simulink model "AFC_FFNN_trainlm_45_45_45_Nor_July_15"  (R2021a)
settings: Solver=ode15s  StartTime=0.0  StopTime=T  MaxStep=.01  RelTol=1e-3
undefined symbols (not defined in the file): AF_sensor_tol, fault_time, fuel_inj_tol, kappa_tol, MAF_sensor_tol, pump_tol, tau_ww_tol, x_gain, x_offset, y_gain, y_offset
libraries: neural x140
(part 2 of 6)

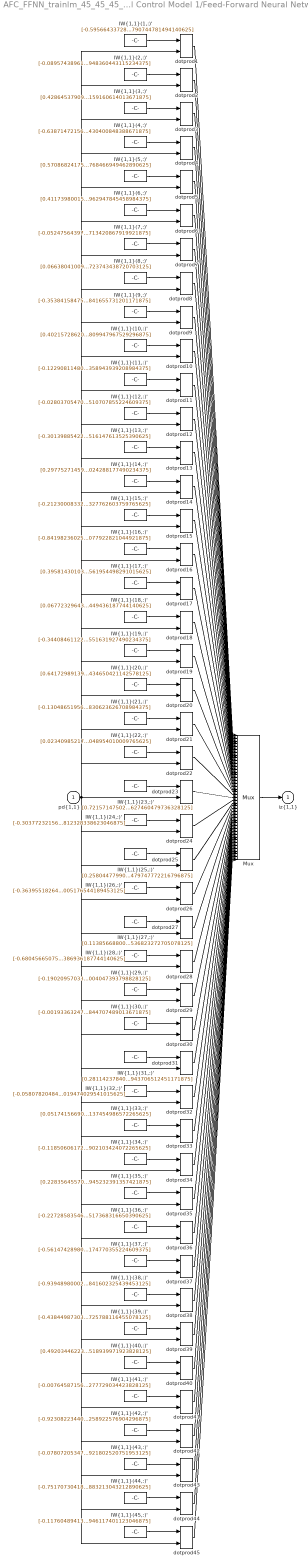
== system AFC_FFNN_trainlm_45_45_45_Nor_July_15/Air Fuel Control Model 1/Feed-Forward Neural Network/Layer 1/IW{1,1} ==
  "pd{1,1}" : Inport  PortDimensions=4
      mask Display: e = 0.06;c1 = [120 230 180]/255;c2 = ([120 230 180]+0)/(256+128);c3 = ([120 230 180]+128)/(256+128);patch([0 1 1 0],[0 0 1 1],c1);patch([0 1 1 1-e 1-e 0+e],[0 0 1 1-e 0+e 0+e],c2);patch([0 0 1 1-e 0+e 0+e],[0 1 1 1-e 1-e 0+e],c3);plot([0 1 1 0 0],[0 0 1 1 0]);
  "IW{1,1}(1,:)'" : Constant  Value=[-0.5956643372825727311692389775998890399932861328125;0.0078851356521167925706095047644339501857757568359375;-0.731583275475554462019545098883099853992462158203125;0.120278687477326062804650064208544790744781494140625]
      mask Display: e = 0.06;c1 = [120 150 230]/255;c2 = ([120 150 230]+0)/383;c3 = ([120 150 230]+128)/383;patch([0 1 1 0],[0 0 1 1],c1);patch([0 1 1 1-e 1-e 0+e],[0 0 1 1-e 0+e 0+e],c2);patch([0 0 1 1-e 0+e 0+e],[0 1 1 1-e 1-e 0+e],c3);plot([0 1 1 0 0],[0 0 1 1 0]);disp('Weights');
  "IW{1,1}(10,:)'" : Constant  Value=[0.40215728620280477567661137072718702256679534912109375;0.215024407178198206924690794039634056389331817626953125;0.2250727041009067119770037379566929303109645843505859375;0.435264136292866143929103373011457733809947967529296875]
      mask Display: e = 0.06;c1 = [120 150 230]/255;c2 = ([120 150 230]+0)/383;c3 = ([120 150 230]+128)/383;patch([0 1 1 0],[0 0 1 1],c1);patch([0 1 1 1-e 1-e 0+e],[0 0 1 1-e 0+e 0+e],c2);patch([0 0 1 1-e 0+e 0+e],[0 1 1 1-e 1-e 0+e],c3);plot([0 1 1 0 0],[0 0 1 1 0]);disp('Weights');
  "IW{1,1}(11,:)'" : Constant  Value=[-0.1229081148035984227817607461474835872650146484375;-0.69490483860332563637030034442432224750518798828125;-0.453944678170142612572135476511903107166290283203125;0.0741787341554722701175705878995358943939208984375]
      mask Display: e = 0.06;c1 = [120 150 230]/255;c2 = ([120 150 230]+0)/383;c3 = ([120 150 230]+128)/383;patch([0 1 1 0],[0 0 1 1],c1);patch([0 1 1 1-e 1-e 0+e],[0 0 1 1-e 0+e 0+e],c2);patch([0 0 1 1-e 0+e 0+e],[0 1 1 1-e 1-e 0+e],c3);plot([0 1 1 0 0],[0 0 1 1 0]);disp('Weights');
  "IW{1,1}(12,:)'" : Constant  Value=[-0.0280370547053085221456125708527906681410968303680419921875;0.0235006232351334908015072500120368204079568386077880859375;-0.99679528598227229441164354284410364925861358642578125;-0.139054055078011662427428518640226684510707855224609375]
      mask Display: e = 0.06;c1 = [120 150 230]/255;c2 = ([120 150 230]+0)/383;c3 = ([120 150 230]+128)/383;patch([0 1 1 0],[0 0 1 1],c1);patch([0 1 1 1-e 1-e 0+e],[0 0 1 1-e 0+e 0+e],c2);patch([0 0 1 1-e 0+e 0+e],[0 1 1 1-e 1-e 0+e],c3);plot([0 1 1 0 0],[0 0 1 1 0]);disp('Weights');
  "IW{1,1}(13,:)'" : Constant  Value=[-0.301398854224746604035800601195660419762134552001953125;0.283042849370989169077716951505863107740879058837890625;0.052267715740464924800701140839009894989430904388427734375;-0.1897669659253120588715546546154655516147613525390625]
      mask Display: e = 0.06;c1 = [120 150 230]/255;c2 = ([120 150 230]+0)/383;c3 = ([120 150 230]+128)/383;patch([0 1 1 0],[0 0 1 1],c1);patch([0 1 1 1-e 1-e 0+e],[0 0 1 1-e 0+e 0+e],c2);patch([0 0 1 1-e 0+e 0+e],[0 1 1 1-e 1-e 0+e],c3);plot([0 1 1 0 0],[0 0 1 1 0]);disp('Weights');
  "IW{1,1}(14,:)'" : Constant  Value=[0.2977527145915799255959655056358315050601959228515625;0.389318770656627621828960172933875583112239837646484375;0.293057371345684547492282945313490927219390869140625;0.2813997438522173322184016797109507024288177490234375]
      mask Display: e = 0.06;c1 = [120 150 230]/255;c2 = ([120 150 230]+0)/383;c3 = ([120 150 230]+128)/383;patch([0 1 1 0],[0 0 1 1],c1);patch([0 1 1 1-e 1-e 0+e],[0 0 1 1-e 0+e 0+e],c2);patch([0 0 1 1-e 0+e 0+e],[0 1 1 1-e 1-e 0+e],c3);plot([0 1 1 0 0],[0 0 1 1 0]);disp('Weights');
  "IW{1,1}(15,:)'" : Constant  Value=[-0.21230008332540395432630475625046528875827789306640625;0.68052922423117545580595333376550115644931793212890625;1.129196089459527652110182316391728818416595458984375;0.38175478396998008268070634585455991327762603759765625]
      mask Display: e = 0.06;c1 = [120 150 230]/255;c2 = ([120 150 230]+0)/383;c3 = ([120 150 230]+128)/383;patch([0 1 1 0],[0 0 1 1],c1);patch([0 1 1 1-e 1-e 0+e],[0 0 1 1-e 0+e 0+e],c2);patch([0 0 1 1-e 0+e 0+e],[0 1 1 1-e 1-e 0+e],c3);plot([0 1 1 0 0],[0 0 1 1 0]);disp('Weights');
  "IW{1,1}(16,:)'" : Constant  Value=[-0.8419823602587410693587344212573952972888946533203125;-0.683631419962078101804081597947515547275543212890625;0.136479567974448823264310703962109982967376708984375;0.424886858909423903440938374842517077922821044921875]
      mask Display: e = 0.06;c1 = [120 150 230]/255;c2 = ([120 150 230]+0)/383;c3 = ([120 150 230]+128)/383;patch([0 1 1 0],[0 0 1 1],c1);patch([0 1 1 1-e 1-e 0+e],[0 0 1 1-e 0+e 0+e],c2);patch([0 0 1 1-e 0+e 0+e],[0 1 1 1-e 1-e 0+e],c3);plot([0 1 1 0 0],[0 0 1 1 0]);disp('Weights');
  "IW{1,1}(17,:)'" : Constant  Value=[0.39581430103202530634831646239035762846469879150390625;0.04913474719346826169452668864323641173541545867919921875;-0.37189361256331088245730143171385861933231353759765625;0.0937071221445386071113858861281187273561954498291015625]
      mask Display: e = 0.06;c1 = [120 150 230]/255;c2 = ([120 150 230]+0)/383;c3 = ([120 150 230]+128)/383;patch([0 1 1 0],[0 0 1 1],c1);patch([0 1 1 1-e 1-e 0+e],[0 0 1 1-e 0+e 0+e],c2);patch([0 0 1 1-e 0+e 0+e],[0 1 1 1-e 1-e 0+e],c3);plot([0 1 1 0 0],[0 0 1 1 0]);disp('Weights');
  "IW{1,1}(18,:)'" : Constant  Value=[0.067723296434411162092459335326566360890865325927734375;0.0782261872747194442201390529589843936264514923095703125;-0.7782064126921157676264328983961604535579681396484375;0.66151523134186407393286799560883082449436187744140625]
      mask Display: e = 0.06;c1 = [120 150 230]/255;c2 = ([120 150 230]+0)/383;c3 = ([120 150 230]+128)/383;patch([0 1 1 0],[0 0 1 1],c1);patch([0 1 1 1-e 1-e 0+e],[0 0 1 1-e 0+e 0+e],c2);patch([0 0 1 1-e 0+e 0+e],[0 1 1 1-e 1-e 0+e],c3);plot([0 1 1 0 0],[0 0 1 1 0]);disp('Weights');
  "IW{1,1}(19,:)'" : Constant  Value=[-0.34408461122719469216235665953718125820159912109375;-0.727276266717437724906858420581556856632232666015625;-0.3469464521698870651533752607065252959728240966796875;-0.8895237546480083690170204135938547551631927490234375]
      mask Display: e = 0.06;c1 = [120 150 230]/255;c2 = ([120 150 230]+0)/383;c3 = ([120 150 230]+128)/383;patch([0 1 1 0],[0 0 1 1],c1);patch([0 1 1 1-e 1-e 0+e],[0 0 1 1-e 0+e 0+e],c2);patch([0 0 1 1-e 0+e 0+e],[0 1 1 1-e 1-e 0+e],c3);plot([0 1 1 0 0],[0 0 1 1 0]);disp('Weights');
  "IW{1,1}(2,:)'" : Constant  Value=[-0.0895743896153724517006367022986523807048797607421875;-0.4974994059611235197593259727000258862972259521484375;-0.556921490563318410949023018474690616130828857421875;-0.1468395671085696019275701473816297948360443115234375]
      mask Display: e = 0.06;c1 = [120 150 230]/255;c2 = ([120 150 230]+0)/383;c3 = ([120 150 230]+128)/383;patch([0 1 1 0],[0 0 1 1],c1);patch([0 1 1 1-e 1-e 0+e],[0 0 1 1-e 0+e 0+e],c2);patch([0 0 1 1-e 0+e 0+e],[0 1 1 1-e 1-e 0+e],c3);plot([0 1 1 0 0],[0 0 1 1 0]);disp('Weights');
  "IW{1,1}(20,:)'" : Constant  Value=[0.64172989139603620056817590011633001267910003662109375;0.241314326391462496967932338520768098533153533935546875;-0.5964552046849258548633088139467872679233551025390625;0.155516258518920758024961514820461161434650421142578125]
      mask Display: e = 0.06;c1 = [120 150 230]/255;c2 = ([120 150 230]+0)/383;c3 = ([120 150 230]+128)/383;patch([0 1 1 0],[0 0 1 1],c1);patch([0 1 1 1-e 1-e 0+e],[0 0 1 1-e 0+e 0+e],c2);patch([0 0 1 1-e 0+e 0+e],[0 1 1 1-e 1-e 0+e],c3);plot([0 1 1 0 0],[0 0 1 1 0]);disp('Weights');
  "IW{1,1}(21,:)'" : Constant  Value=[-0.130486519560841729425959556465386413037776947021484375;0.23962567672372758753596144742914475500583648681640625;1.2471840349032419226205092854797840118408203125;-0.217739378918231751836032117353170178830623626708984375]
      mask Display: e = 0.06;c1 = [120 150 230]/255;c2 = ([120 150 230]+0)/383;c3 = ([120 150 230]+128)/383;patch([0 1 1 0],[0 0 1 1],c1);patch([0 1 1 1-e 1-e 0+e],[0 0 1 1-e 0+e 0+e],c2);patch([0 0 1 1-e 0+e 0+e],[0 1 1 1-e 1-e 0+e],c3);plot([0 1 1 0 0],[0 0 1 1 0]);disp('Weights');
  "IW{1,1}(22,:)'" : Constant  Value=[0.0234098521776516139969448460078638163395226001739501953125;0.01181668668611625915010332477095289505086839199066162109375;0.2319172972597932369520634665605030022561550140380859375;0.053573417723569195791899488767739967443048954010009765625]
      mask Display: e = 0.06;c1 = [120 150 230]/255;c2 = ([120 150 230]+0)/383;c3 = ([120 150 230]+128)/383;patch([0 1 1 0],[0 0 1 1],c1);patch([0 1 1 1-e 1-e 0+e],[0 0 1 1-e 0+e 0+e],c2);patch([0 0 1 1-e 0+e 0+e],[0 1 1 1-e 1-e 0+e],c3);plot([0 1 1 0 0],[0 0 1 1 0]);disp('Weights');
  "IW{1,1}(23,:)'" : Constant  Value=[0.7215714750234367702574900249601341784000396728515625;-0.16108688740140753026253150892443954944610595703125;-0.2450954091114052602051742724142968654632568359375;-0.8883730723524536632140780056943185627460479736328125]
      mask Display: e = 0.06;c1 = [120 150 230]/255;c2 = ([120 150 230]+0)/383;c3 = ([120 150 230]+128)/383;patch([0 1 1 0],[0 0 1 1],c1);patch([0 1 1 1-e 1-e 0+e],[0 0 1 1-e 0+e 0+e],c2);patch([0 0 1 1-e 0+e 0+e],[0 1 1 1-e 1-e 0+e],c3);plot([0 1 1 0 0],[0 0 1 1 0]);disp('Weights');
  "IW{1,1}(24,:)'" : Constant  Value=[-0.303772321561371960729758257002686150372028350830078125;-0.13663066884064811734589284242247231304645538330078125;0.28666251978549073253788037618505768477916717529296875;0.0872318977607193513090777514662477187812328338623046875]
      mask Display: e = 0.06;c1 = [120 150 230]/255;c2 = ([120 150 230]+0)/383;c3 = ([120 150 230]+128)/383;patch([0 1 1 0],[0 0 1 1],c1);patch([0 1 1 1-e 1-e 0+e],[0 0 1 1-e 0+e 0+e],c2);patch([0 0 1 1-e 0+e 0+e],[0 1 1 1-e 1-e 0+e],c3);plot([0 1 1 0 0],[0 0 1 1 0]);disp('Weights');
  "IW{1,1}(25,:)'" : Constant  Value=[0.25804477990530061415341833708225749433040618896484375;-0.1588247856223685416932056568839470855891704559326171875;-0.9527621246937447718750036074197851121425628662109375;0.342543129651466660146041931511717848479747772216796875]
      mask Display: e = 0.06;c1 = [120 150 230]/255;c2 = ([120 150 230]+0)/383;c3 = ([120 150 230]+128)/383;patch([0 1 1 0],[0 0 1 1],c1);patch([0 1 1 1-e 1-e 0+e],[0 0 1 1-e 0+e 0+e],c2);patch([0 0 1 1-e 0+e 0+e],[0 1 1 1-e 1-e 0+e],c3);plot([0 1 1 0 0],[0 0 1 1 0]);disp('Weights');
  "IW{1,1}(26,:)'" : Constant  Value=[-0.3639551826419198388151698964065872132778167724609375;-0.954934179958911055763337571988813579082489013671875;0.9311051108874803805548481250298209488391876220703125;-0.2415869542128252778212527118739672005176544189453125]
      mask Display: e = 0.06;c1 = [120 150 230]/255;c2 = ([120 150 230]+0)/383;c3 = ([120 150 230]+128)/383;patch([0 1 1 0],[0 0 1 1],c1);patch([0 1 1 1-e 1-e 0+e],[0 0 1 1-e 0+e 0+e],c2);patch([0 0 1 1-e 0+e 0+e],[0 1 1 1-e 1-e 0+e],c3);plot([0 1 1 0 0],[0 0 1 1 0]);disp('Weights');
  "IW{1,1}(27,:)'" : Constant  Value=[0.113856688004887851572988211046322248876094818115234375;0.156682594473692093917094325661309994757175445556640625;0.404541877953054129779530967425671406090259552001953125;0.3243492455387972928093631708179600536823272705078125]
      mask Display: e = 0.06;c1 = [120 150 230]/255;c2 = ([120 150 230]+0)/383;c3 = ([120 150 230]+128)/383;patch([0 1 1 0],[0 0 1 1],c1);patch([0 1 1 1-e 1-e 0+e],[0 0 1 1-e 0+e 0+e],c2);patch([0 0 1 1-e 0+e 0+e],[0 1 1 1-e 1-e 0+e],c3);plot([0 1 1 0 0],[0 0 1 1 0]);disp('Weights');
  "IW{1,1}(28,:)'" : Constant  Value=[-0.6804566507554359322540449284133501350879669189453125;-0.9876086455192980562145521616912446916103363037109375;-0.4386537506745231684845975905773229897022247314453125;-0.5337541635500218095700120102264918386936187744140625]
      mask Display: e = 0.06;c1 = [120 150 230]/255;c2 = ([120 150 230]+0)/383;c3 = ([120 150 230]+128)/383;patch([0 1 1 0],[0 0 1 1],c1);patch([0 1 1 1-e 1-e 0+e],[0 0 1 1-e 0+e 0+e],c2);patch([0 0 1 1-e 0+e 0+e],[0 1 1 1-e 1-e 0+e],c3);plot([0 1 1 0 0],[0 0 1 1 0]);disp('Weights');
  "IW{1,1}(29,:)'" : Constant  Value=[-0.19020957033060648111444379537715576589107513427734375;0.0103510998057852292297820184785450692288577556610107421875;2.514854966736393304671537407557480037212371826171875;0.16321702287675876608119551747222431004047393798828125]
      mask Display: e = 0.06;c1 = [120 150 230]/255;c2 = ([120 150 230]+0)/383;c3 = ([120 150 230]+128)/383;patch([0 1 1 0],[0 0 1 1],c1);patch([0 1 1 1-e 1-e 0+e],[0 0 1 1-e 0+e 0+e],c2);patch([0 0 1 1-e 0+e 0+e],[0 1 1 1-e 1-e 0+e],c3);plot([0 1 1 0 0],[0 0 1 1 0]);disp('Weights');
  "IW{1,1}(3,:)'" : Constant  Value=[0.4286453790909512395757019476150162518024444580078125;0.33552739865496128413013821045751683413982391357421875;-0.2115595154244242770413819698660518042743206024169921875;-0.55043277454292194317275743742357008159160614013671875]
      mask Display: e = 0.06;c1 = [120 150 230]/255;c2 = ([120 150 230]+0)/383;c3 = ([120 150 230]+128)/383;patch([0 1 1 0],[0 0 1 1],c1);patch([0 1 1 1-e 1-e 0+e],[0 0 1 1-e 0+e 0+e],c2);patch([0 0 1 1-e 0+e 0+e],[0 1 1 1-e 1-e 0+e],c3);plot([0 1 1 0 0],[0 0 1 1 0]);disp('Weights');
  "IW{1,1}(30,:)'" : Constant  Value=[-0.00193363247180133868141638231463730335235595703125;0.1267069804364975293964334923657588660717010498046875;0.1556430626833267272246530410484410822391510009765625;-0.548593431939991216239604909787885844707489013671875]
      mask Display: e = 0.06;c1 = [120 150 230]/255;c2 = ([120 150 230]+0)/383;c3 = ([120 150 230]+128)/383;patch([0 1 1 0],[0 0 1 1],c1);patch([0 1 1 1-e 1-e 0+e],[0 0 1 1-e 0+e 0+e],c2);patch([0 0 1 1-e 0+e 0+e],[0 1 1 1-e 1-e 0+e],c3);plot([0 1 1 0 0],[0 0 1 1 0]);disp('Weights');
  "IW{1,1}(31,:)'" : Constant  Value=[0.2811423784052606844596766677568666636943817138671875;0.57790938879531894567520566852181218564510345458984375;-0.9063653540192044832934925580048002302646636962890625;0.5131888068818895032308091685990802943706512451171875]
      mask Display: e = 0.06;c1 = [120 150 230]/255;c2 = ([120 150 230]+0)/383;c3 = ([120 150 230]+128)/383;patch([0 1 1 0],[0 0 1 1],c1);patch([0 1 1 1-e 1-e 0+e],[0 0 1 1-e 0+e 0+e],c2);patch([0 0 1 1-e 0+e 0+e],[0 1 1 1-e 1-e 0+e],c3);plot([0 1 1 0 0],[0 0 1 1 0]);disp('Weights');
  "IW{1,1}(32,:)'" : Constant  Value=[-0.058078204842097129467770599831055733375251293182373046875;-0.001563164818252172315327097606996176182292401790618896484375;0.82613033699437432577639128794544376432895660400390625;0.1453053847708275780892250850229174830019474029541015625]
      mask Display: e = 0.06;c1 = [120 150 230]/255;c2 = ([120 150 230]+0)/383;c3 = ([120 150 230]+128)/383;patch([0 1 1 0],[0 0 1 1],c1);patch([0 1 1 1-e 1-e 0+e],[0 0 1 1-e 0+e 0+e],c2);patch([0 0 1 1-e 0+e 0+e],[0 1 1 1-e 1-e 0+e],c3);plot([0 1 1 0 0],[0 0 1 1 0]);disp('Weights');
  "IW{1,1}(33,:)'" : Constant  Value=[0.05174156690815133463612340847248560748994350433349609375;0.417236200443662996750759930364438332617282867431640625;0.28576353561735334807281105895526707172393798828125;-0.2301783314639698208026175052509643137454986572265625]
      mask Display: e = 0.06;c1 = [120 150 230]/255;c2 = ([120 150 230]+0)/383;c3 = ([120 150 230]+128)/383;patch([0 1 1 0],[0 0 1 1],c1);patch([0 1 1 1-e 1-e 0+e],[0 0 1 1-e 0+e 0+e],c2);patch([0 0 1 1-e 0+e 0+e],[0 1 1 1-e 1-e 0+e],c3);plot([0 1 1 0 0],[0 0 1 1 0]);disp('Weights');
  "IW{1,1}(34,:)'" : Constant  Value=[-0.11850606172833634543994918431053520180284976959228515625;0.64849251750362368884594843621016480028629302978515625;-0.66071595290289197865973847001441754400730133056640625;-0.08370208249480794171493158728480921126902103424072265625]
      mask Display: e = 0.06;c1 = [120 150 230]/255;c2 = ([120 150 230]+0)/383;c3 = ([120 150 230]+128)/383;patch([0 1 1 0],[0 0 1 1],c1);patch([0 1 1 1-e 1-e 0+e],[0 0 1 1-e 0+e 0+e],c2);patch([0 0 1 1-e 0+e 0+e],[0 1 1 1-e 1-e 0+e],c3);plot([0 1 1 0 0],[0 0 1 1 0]);disp('Weights');
  "IW{1,1}(35,:)'" : Constant  Value=[0.22835645570773610568693356981384567916393280029296875;-0.54905905338665250692287145284353755414485931396484375;-0.89228427011588318240598027841770090162754058837890625;0.1158953695663818006522660652990452945232391357421875]
      mask Display: e = 0.06;c1 = [120 150 230]/255;c2 = ([120 150 230]+0)/383;c3 = ([120 150 230]+128)/383;patch([0 1 1 0],[0 0 1 1],c1);patch([0 1 1 1-e 1-e 0+e],[0 0 1 1-e 0+e 0+e],c2);patch([0 0 1 1-e 0+e 0+e],[0 1 1 1-e 1-e 0+e],c3);plot([0 1 1 0 0],[0 0 1 1 0]);disp('Weights');
  "IW{1,1}(36,:)'" : Constant  Value=[-0.2272858354609279540881061620893888175487518310546875;-0.4763666279626981303607635709340684115886688232421875;0.51951620528753483796435830299742519855499267578125;-0.564515386968702959080701475613750517368316650390625]
      mask Display: e = 0.06;c1 = [120 150 230]/255;c2 = ([120 150 230]+0)/383;c3 = ([120 150 230]+128)/383;patch([0 1 1 0],[0 0 1 1],c1);patch([0 1 1 1-e 1-e 0+e],[0 0 1 1-e 0+e 0+e],c2);patch([0 0 1 1-e 0+e 0+e],[0 1 1 1-e 1-e 0+e],c3);plot([0 1 1 0 0],[0 0 1 1 0]);disp('Weights');
  "IW{1,1}(37,:)'" : Constant  Value=[-0.5614742898029103645995974147808738052845001220703125;-0.29126643634214133271598257124423980712890625;0.152044548675759561007225784123875200748443603515625;-0.59448016906409151260959333740174770355224609375]
      mask Display: e = 0.06;c1 = [120 150 230]/255;c2 = ([120 150 230]+0)/383;c3 = ([120 150 230]+128)/383;patch([0 1 1 0],[0 0 1 1],c1);patch([0 1 1 1-e 1-e 0+e],[0 0 1 1-e 0+e 0+e],c2);patch([0 0 1 1-e 0+e 0+e],[0 1 1 1-e 1-e 0+e],c3);plot([0 1 1 0 0],[0 0 1 1 0]);disp('Weights');
  "IW{1,1}(38,:)'" : Constant  Value=[-0.939489800028924459951440439908765256404876708984375;0.4051451785018820306305542544578202068805694580078125;-0.861338665941364656220002871123142540454864501953125;-0.52987044420598294891533441841602325439453125]
      mask Display: e = 0.06;c1 = [120 150 230]/255;c2 = ([120 150 230]+0)/383;c3 = ([120 150 230]+128)/383;patch([0 1 1 0],[0 0 1 1],c1);patch([0 1 1 1-e 1-e 0+e],[0 0 1 1-e 0+e 0+e],c2);patch([0 0 1 1-e 0+e 0+e],[0 1 1 1-e 1-e 0+e],c3);plot([0 1 1 0 0],[0 0 1 1 0]);disp('Weights');
  "IW{1,1}(39,:)'" : Constant  Value=[-0.438449873032815184981103584505035541951656341552734375;0.82358882068447314406256509755621664226055145263671875;-0.054224785744120963804082435899545089341700077056884765625;0.52110169311764586996815751263056881725788116455078125]
      mask Display: e = 0.06;c1 = [120 150 230]/255;c2 = ([120 150 230]+0)/383;c3 = ([120 150 230]+128)/383;patch([0 1 1 0],[0 0 1 1],c1);patch([0 1 1 1-e 1-e 0+e],[0 0 1 1-e 0+e 0+e],c2);patch([0 0 1 1-e 0+e 0+e],[0 1 1 1-e 1-e 0+e],c3);plot([0 1 1 0 0],[0 0 1 1 0]);disp('Weights');
  "IW{1,1}(4,:)'" : Constant  Value=[-0.6387147215604758176965560778626240789890289306640625;-0.1557107718810311070001262123696506023406982421875;-0.64377405270552490179625237942673265933990478515625;-0.8954322416204518741977835816214792430400848388671875]
      mask Display: e = 0.06;c1 = [120 150 230]/255;c2 = ([120 150 230]+0)/383;c3 = ([120 150 230]+128)/383;patch([0 1 1 0],[0 0 1 1],c1);patch([0 1 1 1-e 1-e 0+e],[0 0 1 1-e 0+e 0+e],c2);patch([0 0 1 1-e 0+e 0+e],[0 1 1 1-e 1-e 0+e],c3);plot([0 1 1 0 0],[0 0 1 1 0]);disp('Weights');
  "IW{1,1}(40,:)'" : Constant  Value=[0.492034462236722702765945314240525476634502410888671875;-0.1777275222817087663162993749210727401077747344970703125;0.0099231706383438623986226190254456014372408390045166015625;-0.5146204597120729307135889030178077518939971923828125]
      mask Display: e = 0.06;c1 = [120 150 230]/255;c2 = ([120 150 230]+0)/383;c3 = ([120 150 230]+128)/383;patch([0 1 1 0],[0 0 1 1],c1);patch([0 1 1 1-e 1-e 0+e],[0 0 1 1-e 0+e 0+e],c2);patch([0 0 1 1-e 0+e 0+e],[0 1 1 1-e 1-e 0+e],c3);plot([0 1 1 0 0],[0 0 1 1 0]);disp('Weights');
  "IW{1,1}(41,:)'" : Constant  Value=[-0.007645871561652416679988331082995500764809548854827880859375;0.035310008323311013744838504635481513105332851409912109375;0.669218883200376257747166164335794746875762939453125;-0.29644770762242089734428418523748405277729034423828125]
      mask Display: e = 0.06;c1 = [120 150 230]/255;c2 = ([120 150 230]+0)/383;c3 = ([120 150 230]+128)/383;patch([0 1 1 0],[0 0 1 1],c1);patch([0 1 1 1-e 1-e 0+e],[0 0 1 1-e 0+e 0+e],c2);patch([0 0 1 1-e 0+e 0+e],[0 1 1 1-e 1-e 0+e],c3);plot([0 1 1 0 0],[0 0 1 1 0]);disp('Weights');
  "IW{1,1}(42,:)'" : Constant  Value=[-0.9230822344099307574794011088670231401920318603515625;0.0345640338353359055645341868512332439422607421875;-0.8821807032780721868903128779493272304534912109375;-0.016831332291136202883308214950375258922576904296875]
      mask Display: e = 0.06;c1 = [120 150 230]/255;c2 = ([120 150 230]+0)/383;c3 = ([120 150 230]+128)/383;patch([0 1 1 0],[0 0 1 1],c1);patch([0 1 1 1-e 1-e 0+e],[0 0 1 1-e 0+e 0+e],c2);patch([0 0 1 1-e 0+e 0+e],[0 1 1 1-e 1-e 0+e],c3);plot([0 1 1 0 0],[0 0 1 1 0]);disp('Weights');
  "IW{1,1}(43,:)'" : Constant  Value=[-0.0780720534746517369484308801474981009960174560546875;-0.76974465630501498480953159742057323455810546875;0.1214981365683154290735501490416936576366424560546875;-0.54355568559331590705596681800670921802520751953125]
      mask Display: e = 0.06;c1 = [120 150 230]/255;c2 = ([120 150 230]+0)/383;c3 = ([120 150 230]+128)/383;patch([0 1 1 0],[0 0 1 1],c1);patch([0 1 1 1-e 1-e 0+e],[0 0 1 1-e 0+e 0+e],c2);patch([0 0 1 1-e 0+e 0+e],[0 1 1 1-e 1-e 0+e],c3);plot([0 1 1 0 0],[0 0 1 1 0]);disp('Weights');
  "IW{1,1}(44,:)'" : Constant  Value=[-0.751707304187491320845992959220893681049346923828125;0.198396436014707688855196465738117694854736328125;0.7254043262583362849937884675455279648303985595703125;-0.918083848242825073526773849152959883213043212890625]
      mask Display: e = 0.06;c1 = [120 150 230]/255;c2 = ([120 150 230]+0)/383;c3 = ([120 150 230]+128)/383;patch([0 1 1 0],[0 0 1 1],c1);patch([0 1 1 1-e 1-e 0+e],[0 0 1 1-e 0+e 0+e],c2);patch([0 0 1 1-e 0+e 0+e],[0 1 1 1-e 1-e 0+e],c3);plot([0 1 1 0 0],[0 0 1 1 0]);disp('Weights');
  "IW{1,1}(45,:)'" : Constant  Value=[-0.11760489413344958620211144761924515478312969207763671875;-0.06724246508251256748689428377474541775882244110107421875;1.716790267288401228285010802210308611392974853515625;0.138135284928623203182240786190959624946117401123046875]
      mask Display: e = 0.06;c1 = [120 150 230]/255;c2 = ([120 150 230]+0)/383;c3 = ([120 150 230]+128)/383;patch([0 1 1 0],[0 0 1 1],c1);patch([0 1 1 1-e 1-e 0+e],[0 0 1 1-e 0+e 0+e],c2);patch([0 0 1 1-e 0+e 0+e],[0 1 1 1-e 1-e 0+e],c3);plot([0 1 1 0 0],[0 0 1 1 0]);disp('Weights');
  "IW{1,1}(5,:)'" : Constant  Value=[0.57086824175524986113572367685264907777309417724609375;0.42698472150594624086039630128652788698673248291015625;-0.911692582119400629636629673768766224384307861328125;0.343660323975889137049222199493669904768466949462890625]
      mask Display: e = 0.06;c1 = [120 150 230]/255;c2 = ([120 150 230]+0)/383;c3 = ([120 150 230]+128)/383;patch([0 1 1 0],[0 0 1 1],c1);patch([0 1 1 1-e 1-e 0+e],[0 0 1 1-e 0+e 0+e],c2);patch([0 0 1 1-e 0+e 0+e],[0 1 1 1-e 1-e 0+e],c3);plot([0 1 1 0 0],[0 0 1 1 0]);disp('Weights');
  "IW{1,1}(6,:)'" : Constant  Value=[0.411739800154247548302777204298763535916805267333984375;0.422359992132983197432594124620663933455944061279296875;0.87224581114104549062204796427977271378040313720703125;0.509079625495759469089307458489201962947845458984375]
      mask Display: e = 0.06;c1 = [120 150 230]/255;c2 = ([120 150 230]+0)/383;c3 = ([120 150 230]+128)/383;patch([0 1 1 0],[0 0 1 1],c1);patch([0 1 1 1-e 1-e 0+e],[0 0 1 1-e 0+e 0+e],c2);patch([0 0 1 1-e 0+e 0+e],[0 1 1 1-e 1-e 0+e],c3);plot([0 1 1 0 0],[0 0 1 1 0]);disp('Weights');
  "IW{1,1}(7,:)'" : Constant  Value=[-0.052475643970241188374092899948664125986397266387939453125;-0.00307760460118986813038421956889578723348677158355712890625;0.36598350317306316270560273551382124423980712890625;0.00183832148789884216970313968175787522341124713420867919921875]
      mask Display: e = 0.06;c1 = [120 150 230]/255;c2 = ([120 150 230]+0)/383;c3 = ([120 150 230]+128)/383;patch([0 1 1 0],[0 0 1 1],c1);patch([0 1 1 1-e 1-e 0+e],[0 0 1 1-e 0+e 0+e],c2);patch([0 0 1 1-e 0+e 0+e],[0 1 1 1-e 1-e 0+e],c3);plot([0 1 1 0 0],[0 0 1 1 0]);disp('Weights');
  "IW{1,1}(8,:)'" : Constant  Value=[0.06638041009858490493211746752422186546027660369873046875;0.08490616339429089831636332519337884150445461273193359375;0.7228527644966344922750067780725657939910888671875;0.09808997951294513850672984744960558600723743438720703125]
      mask Display: e = 0.06;c1 = [120 150 230]/255;c2 = ([120 150 230]+0)/383;c3 = ([120 150 230]+128)/383;patch([0 1 1 0],[0 0 1 1],c1);patch([0 1 1 1-e 1-e 0+e],[0 0 1 1-e 0+e 0+e],c2);patch([0 0 1 1-e 0+e 0+e],[0 1 1 1-e 1-e 0+e],c3);plot([0 1 1 0 0],[0 0 1 1 0]);disp('Weights');
  "IW{1,1}(9,:)'" : Constant  Value=[-0.3538415847598563868103838103706948459148406982421875;-0.114457947078893951253775185250560753047466278076171875;0.45418337183023693715000490556121803820133209228515625;-0.78880532703290995311107280940632335841655731201171875]
      mask Display: e = 0.06;c1 = [120 150 230]/255;c2 = ([120 150 230]+0)/383;c3 = ([120 150 230]+128)/383;patch([0 1 1 0],[0 0 1 1],c1);patch([0 1 1 1-e 1-e 0+e],[0 0 1 1-e 0+e 0+e],c2);patch([0 0 1 1-e 0+e 0+e],[0 1 1 1-e 1-e 0+e],c3);plot([0 1 1 0 0],[0 0 1 1 0]);disp('Weights');
  Mux : Mux  Inputs=45
      mask Display: e = 0.06;c1 = [120 150 230]/255;c2 = ([120 150 230]+0)/383;c3 = ([120 150 230]+128)/383;patch([0 1 1 0],[0 0 1 1],c1);patch([0 1 1 1-e 1-e 0+e],[0 0 1 1-e 0+e 0+e],c2);patch([0 0 1 1-e 0+e 0+e],[0 1 1 1-e 1-e 0+e],c3);plot([0 1 1 0 0],[0 0 1 1 0]);disp('Mux');
  dotprod{1..45} (45 alike) : neural/Weight Functions/dotprod
  "iz{1,1}" : Outport
      mask Display: e = 0.06;c1 = [120 230 180]/255;c2 = ([120 230 180]+0)/(256+128);c3 = ([120 230 180]+128)/(256+128);patch([0 1 1 0],[0 0 1 1],c1);patch([0 1 1 1-e 1-e 0+e],[0 0 1 1-e 0+e 0+e],c2);patch([0 0 1 1-e 0+e 0+e],[0 1 1 1-e 1-e 0+e],c3);plot([0 1 1 0 0],[0 0 1 1 0]);
  wires:
  Mux/1 -> "iz{1,1}"/1
  dotprod45/1 -> Mux/45
  "IW{1,1}(45,:)'"/1 -> dotprod45/1
  dotprod44/1 -> Mux/44
  "IW{1,1}(44,:)'"/1 -> dotprod44/1
  dotprod43/1 -> Mux/43
  "IW{1,1}(43,:)'"/1 -> dotprod43/1
  dotprod42/1 -> Mux/42
  "IW{1,1}(42,:)'"/1 -> dotprod42/1
  dotprod41/1 -> Mux/41
  "IW{1,1}(41,:)'"/1 -> dotprod41/1
  dotprod40/1 -> Mux/40
  "IW{1,1}(40,:)'"/1 -> dotprod40/1
  dotprod39/1 -> Mux/39
  "IW{1,1}(39,:)'"/1 -> dotprod39/1
  dotprod38/1 -> Mux/38
  "IW{1,1}(38,:)'"/1 -> dotprod38/1
  dotprod37/1 -> Mux/37
  "IW{1,1}(37,:)'"/1 -> dotprod37/1
  dotprod36/1 -> Mux/36
  "IW{1,1}(36,:)'"/1 -> dotprod36/1
  dotprod35/1 -> Mux/35
  "IW{1,1}(35,:)'"/1 -> dotprod35/1
  dotprod34/1 -> Mux/34
  "IW{1,1}(34,:)'"/1 -> dotprod34/1
  dotprod33/1 -> Mux/33
  "IW{1,1}(33,:)'"/1 -> dotprod33/1
  dotprod32/1 -> Mux/32
  "IW{1,1}(32,:)'"/1 -> dotprod32/1
  dotprod31/1 -> Mux/31
  "IW{1,1}(31,:)'"/1 -> dotprod31/1
  dotprod30/1 -> Mux/30
  "IW{1,1}(30,:)'"/1 -> dotprod30/1
  dotprod29/1 -> Mux/29
  "IW{1,1}(29,:)'"/1 -> dotprod29/1
  dotprod28/1 -> Mux/28
  "IW{1,1}(28,:)'"/1 -> dotprod28/1
  dotprod27/1 -> Mux/27
  "IW{1,1}(27,:)'"/1 -> dotprod27/1
  dotprod26/1 -> Mux/26
  "IW{1,1}(26,:)'"/1 -> dotprod26/1
  dotprod25/1 -> Mux/25
  "IW{1,1}(25,:)'"/1 -> dotprod25/1
  dotprod24/1 -> Mux/24
  "IW{1,1}(24,:)'"/1 -> dotprod24/1
  dotprod23/1 -> Mux/23
  "IW{1,1}(23,:)'"/1 -> dotprod23/1
  dotprod22/1 -> Mux/22
  "IW{1,1}(22,:)'"/1 -> dotprod22/1
  dotprod21/1 -> Mux/21
  "IW{1,1}(21,:)'"/1 -> dotprod21/1
  dotprod20/1 -> Mux/20
  "IW{1,1}(20,:)'"/1 -> dotprod20/1
  dotprod19/1 -> Mux/19
  "IW{1,1}(19,:)'"/1 -> dotprod19/1
  dotprod18/1 -> Mux/18
  "IW{1,1}(18,:)'"/1 -> dotprod18/1
  dotprod17/1 -> Mux/17
  "IW{1,1}(17,:)'"/1 -> dotprod17/1
  dotprod16/1 -> Mux/16
  "IW{1,1}(16,:)'"/1 -> dotprod16/1
  dotprod15/1 -> Mux/15
  "IW{1,1}(15,:)'"/1 -> dotprod15/1
  dotprod14/1 -> Mux/14
  "IW{1,1}(14,:)'"/1 -> dotprod14/1
  dotprod13/1 -> Mux/13
  "IW{1,1}(13,:)'"/1 -> dotprod13/1
  dotprod12/1 -> Mux/12
  "IW{1,1}(12,:)'"/1 -> dotprod12/1
  dotprod11/1 -> Mux/11
  "IW{1,1}(11,:)'"/1 -> dotprod11/1
  dotprod10/1 -> Mux/10
  "IW{1,1}(10,:)'"/1 -> dotprod10/1
  dotprod9/1 -> Mux/9
  "IW{1,1}(9,:)'"/1 -> dotprod9/1
  dotprod8/1 -> Mux/8
  "IW{1,1}(8,:)'"/1 -> dotprod8/1
  dotprod7/1 -> Mux/7
  "IW{1,1}(7,:)'"/1 -> dotprod7/1
  dotprod6/1 -> Mux/6
  "IW{1,1}(6,:)'"/1 -> dotprod6/1
  dotprod5/1 -> Mux/5
  "IW{1,1}(5,:)'"/1 -> dotprod5/1
  dotprod4/1 -> Mux/4
  "IW{1,1}(4,:)'"/1 -> dotprod4/1
  dotprod3/1 -> Mux/3
  "IW{1,1}(3,:)'"/1 -> dotprod3/1
  dotprod2/1 -> Mux/2
  "IW{1,1}(2,:)'"/1 -> dotprod2/1
  dotprod1/1 -> Mux/1
  "pd{1,1}"/1 -> dotprod45/2, dotprod44/2, dotprod43/2, dotprod42/2, dotprod41/2, dotprod40/2, dotprod39/2, dotprod38/2, dotprod37/2, dotprod36/2, dotprod35/2, dotprod34/2, dotprod33/2, dotprod32/2, dotprod31/2, dotprod30/2, dotprod29/2, dotprod28/2, dotprod27/2, dotprod26/2, dotprod25/2, dotprod24/2, dotprod23/2, dotprod22/2, dotprod21/2, dotprod20/2, dotprod19/2, dotprod18/2, dotprod17/2, dotprod16/2, dotprod15/2, dotprod14/2, dotprod13/2, dotprod12/2, dotprod11/2, dotprod10/2, dotprod9/2, dotprod8/2, dotprod7/2, dotprod6/2, dotprod5/2, dotprod4/2, dotprod3/2, dotprod2/2, dotprod1/2
  "IW{1,1}(1,:)'"/1 -> dotprod1/1

== system AFC_FFNN_trainlm_45_45_45_Nor_July_15/Air Fuel Control Model 1/Feed-Forward Neural Network/Layer 2/Delays 1 ==
  "p{2}" : Inport  PortDimensions=45
      mask Display: e = 0.06;c1 = [120 230 180]/255;c2 = ([120 230 180]+0)/(256+128);c3 = ([120 230 180]+128)/(256+128);patch([0 1 1 0],[0 0 1 1],c1);patch([0 1 1 1-e 1-e 0+e],[0 0 1 1-e 0+e 0+e],c2);patch([0 0 1 1-e 0+e 0+e],[0 1 1 1-e 1-e 0+e],c3);plot([0 1 1 0 0],[0 0 1 1 0]);
  mux : Mux  Inputs=1
      mask Display: e = 0.06;c1 = [120 150 230]/255;c2 = ([120 150 230]+0)/383;c3 = ([120 150 230]+128)/383;patch([0 1 1 0],[0 0 1 1],c1);patch([0 1 1 1-e 1-e 0+e],[0 0 1 1-e 0+e 0+e],c2);patch([0 0 1 1-e 0+e 0+e],[0 1 1 1-e 1-e 0+e],c3);plot([0 1 1 0 0],[0 0 1 1 0]);disp('Mux')
  "pd{2,1}" : Outport
      mask Display: e = 0.06;c1 = [120 230 180]/255;c2 = ([120 230 180]+0)/(256+128);c3 = ([120 230 180]+128)/(256+128);patch([0 1 1 0],[0 0 1 1],c1);patch([0 1 1 1-e 1-e 0+e],[0 0 1 1-e 0+e 0+e],c2);patch([0 0 1 1-e 0+e 0+e],[0 1 1 1-e 1-e 0+e],c3);plot([0 1 1 0 0],[0 0 1 1 0]);
  wires:
  mux/1 -> "pd{2,1}"/1
  "p{2}"/1 -> mux/1
